simulink model "QPSK_System_Over_AWGN_Channel"  (R2025b)
settings: Solver=VariableStepAuto  StartTime=0.0  StopTime=inf  RelTol=1e-3
values from neighbouring files (symbols this model uses):
  EbNo_dB = EbNo_values(k)    [Sweep_SNR_BPSK.m]    (also in Sweep_SNR_QPSK.m)
libraries: simulink x3, commfilt2 x2, commchan3 x1, commrandsrc3 x1, commsink2 x1
settings Model: Creator=Bharath Kumar Reddy  LastModifiedBy=Bharath Kumar Reddy

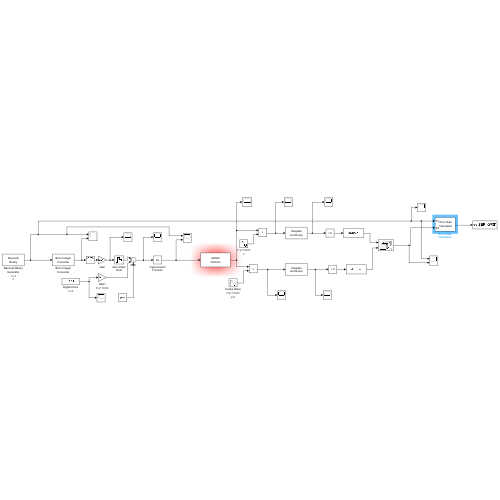
[thumbnail: Simulink's stored preview of the top-level diagram]
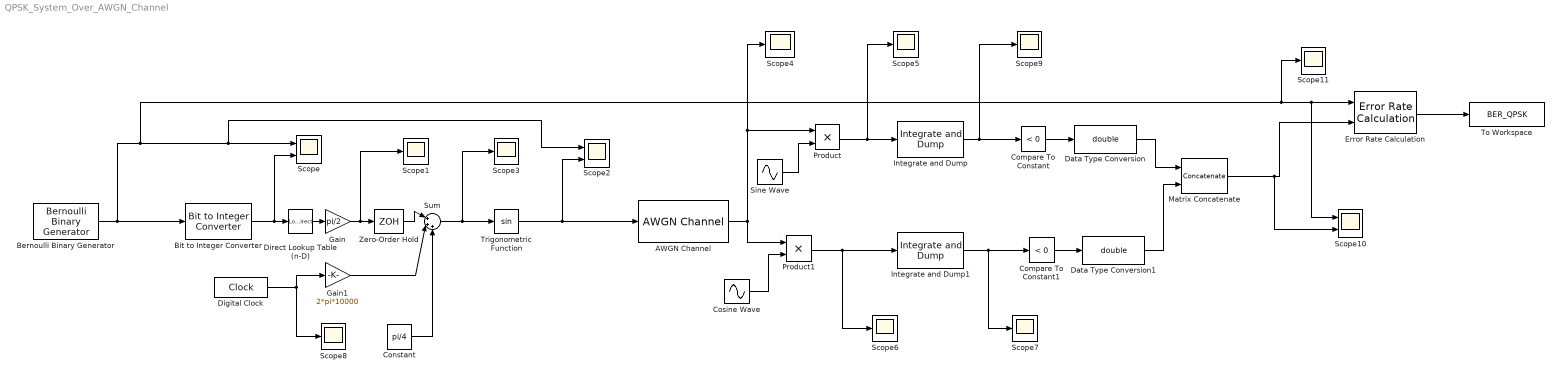
== system QPSK_System_Over_AWGN_Channel ==
  AWGN Channel : commchan3/AWGN Channel  LegacyMode=off  NoiseMethod="Signal to noise ratio  (Es/No)"  noiseMode="Signal to noise ratio  (SNR)"  EbNo=10  EsNo=EbNo_dB + 10*log10(2)  SNR=10  BitsPerSymbol=1  SignalPower=0.5  SpecifySymbolPeriod=off  SamplesPerSymbol=200  SymbolPeriod=1  VarianceSource=Parameter  Variance=1  RandomStream=Global stream  Seed=67  SimulateUsing=Code generation
  Bernoulli Binary Generator : commrandsrc3/Bernoulli Binary Generator  ProbabilityOfZero=0.5  SeedSource=Auto  Seed=0  SampleTime=1e-4  SamplesPerFrame=2  OutputDataType=double  SimulateUsing=Interpreted execution
      settings: AttributesFormatString=|
      | %<SampleTime>
      | %<SamplesPerFrame>
  Bit to Integer Converter : simulink/Logic and Bit Operations/Bit to Integer Converter  nbits=2  bitOrder=MSB first  signedOutputValues=Unsigned  outDtype=Inherit via internal rule  outDtypeSigned=Inherit via internal rule
  Compare To Constant : simulink/Logic and Bit Operations/Compare To Constant  relop=<  const=0  OutDataTypeStr=boolean
  Compare To Constant1 : simulink/Logic and Bit Operations/Compare To Constant  relop=<  const=0  OutDataTypeStr=boolean
  Constant : Constant  Value=pi/4
  Cosine Wave : Sin  Amplitude=2  Frequency=2*pi*10000  Phase=pi/2  SampleTime=1e-6
      settings: AttributesFormatString=|
      | %<Frequency>
      | %<Phase>
  Data Type Conversion : DataTypeConversion  OutDataTypeStr=double  SaturateOnIntegerOverflow=off  RndMeth=Floor
  Data Type Conversion1 : DataTypeConversion  OutDataTypeStr=double  SaturateOnIntegerOverflow=off  RndMeth=Floor
  Digital Clock : DigitalClock  SampleTime=1e-6
      settings: AttributesFormatString=%<SampleTime>
  Direct Lookup Table (n-D) : LookupNDDirect  NumberOfTableDimensions=1  Table=[0 3 1 2]
  Error Rate Calculation : commsink2/Error Rate Calculation  N=2  st_delay=0  cp_mode=Entire frame  subframe=[]  PMode=Port  WsName=ErrorVec  RsMode2=off  stop=on  numErr=100  maxBits=1e4
  Gain : Gain  Gain=pi/2
  Gain1 : Gain  Gain=2*pi*10000
      settings: AttributesFormatString=%<Gain>
  Integrate and Dump : commfilt2/Integrate and Dump  obssamples=200  offsetsamples=0  nodump=off  roundingMode=Floor  overflowMode=off  outputDataTypeStr=Inherit: Same as accumulator  outputLastDataTypeStr=Inherit: Same as accumulator
  Integrate and Dump1 : commfilt2/Integrate and Dump  obssamples=200  offsetsamples=0  nodump=off  roundingMode=Floor  overflowMode=off  outputDataTypeStr=Inherit: Same as accumulator  outputLastDataTypeStr=Inherit: Same as accumulator
  Matrix Concatenate : Concatenate  Mode=Multidimensional array
  Product : Product
  Product1 : Product
  Scope : Scope  NumInputPorts=2
      settings: ActiveDisplayYMinimum=-0.37499999999999989  ActiveDisplayYMaximum=3.375
  Scope{1,3..9,11} (9 alike) : Scope
      Scope1 settings: ActiveDisplayYMinimum=-1  ActiveDisplayYMaximum=1
      Scope11 settings: ActiveDisplayYMinimum=-1  ActiveDisplayYMaximum=1  DataLoggingVariableName=ScopeData11
      Scope3 settings: ActiveDisplayYMinimum=-1  ActiveDisplayYMaximum=1  DataLoggingVariableName=ScopeData3
      Scope4 settings: ActiveDisplayYMinimum=-1.2792340034529786  ActiveDisplayYMaximum=1.385277866499266  DataLoggingVariableName=ScopeData4
      Scope5 settings: ActiveDisplayYMinimum=-1  ActiveDisplayYMaximum=1  DataLoggingVariableName=ScopeData5
      Scope6 settings: ActiveDisplayYMinimum=-1  ActiveDisplayYMaximum=1  DataLoggingVariableName=ScopeData6
      Scope7 settings: ActiveDisplayYMinimum=-1  ActiveDisplayYMaximum=1  DataLoggingVariableName=ScopeData7
      Scope8 settings: ActiveDisplayYMinimum=-1  ActiveDisplayYMaximum=1  DataLoggingVariableName=ScopeData8
      Scope9 settings: ActiveDisplayYMinimum=-1  ActiveDisplayYMaximum=1  DataLoggingVariableName=ScopeData9
  Scope10 : Scope  NumInputPorts=2
      settings: ActiveDisplayYMinimum=-0.37499999999999989  ActiveDisplayYMaximum=3.375  DataLoggingVariableName=ScopeData10
  Scope2 : Scope  NumInputPorts=2
      settings: ActiveDisplayYMinimum=-1.2494448804131013  ActiveDisplayYMaximum=1.2499383200459002  DataLoggingVariableName=ScopeData2
  Sine Wave : Sin  Amplitude=2  Frequency=2*pi*10000  SampleTime=1e-6
      settings: AttributesFormatString=|
      | %<Frequency>
      | %<Phase>
  Sum : Sum  Inputs=|+++
  To Workspace : ToWorkspace  VariableName=BER_QPSK  SaveFormat=Timeseries  SampleTime=-1
  Trigonometric Function : Trigonometry
  Zero-Order Hold : ZeroOrderHold  SampleTime=1e-4
  wires:
  Bit to Integer Converter/1 -> Direct Lookup Table (n-D)/1, Scope/2
  Gain1/1 -> Sum/2
  Sum/1 -> Scope3/1, Trigonometric Function/1
  Trigonometric Function/1 -> AWGN Channel/1, Scope2/2
  Digital Clock/1 -> Scope8/1, Gain1/1
  AWGN Channel/1 -> Scope4/1, Product/1, Product1/1
  Sine Wave/1 -> Product/2
  Product/1 -> Integrate and Dump/1, Scope5/1
  Cosine Wave/1 -> Product1/2
  Product1/1 -> Integrate and Dump1/1, Scope6/1
  Gain/1 -> Zero-Order Hold/1, Scope1/1
  Zero-Order Hold/1 -> Sum/1
  Integrate and Dump/1 -> Compare To Constant/1, Scope9/1
  Constant/1 -> Sum/3
  Integrate and Dump1/1 -> Compare To Constant1/1, Scope7/1
  Compare To Constant/1 -> Data Type Conversion/1
  Compare To Constant1/1 -> Data Type Conversion1/1
  Data Type Conversion/1 -> Matrix Concatenate/1
  Data Type Conversion1/1 -> Matrix Concatenate/2
  Bernoulli Binary Generator/1 -> Bit to Integer Converter/1, Scope11/1, Error Rate Calculation/1, Scope10/1, Scope2/1, Scope/1
  Error Rate Calculation/1 -> To Workspace/1
  Direct Lookup Table (n-D)/1 -> Gain/1
  Matrix Concatenate/1 -> Scope10/2, Error Rate Calculation/2
